simulink model "scara_stepper"  (R2026a)
settings: Solver=FixedStepDiscrete  StopTime=scara_ref.t(end)  FixedStep=scara_p.dt
InitFcn:
  | addpath(fileparts(fileparts(fileparts(get_param(bdroot,'FileName'))))); startup_scara(); if ~exist('scara_steps_signal','var') || ~exist('scara_ref','var') || ~isfield(scara_ref,'steps'), scara_setup('flower'); end
undefined symbols (not defined in the file): scara_p, scara_q0, scara_ref
libraries: simulink x14
settings Model: Creator=vutua  LastModifiedBy=vutua

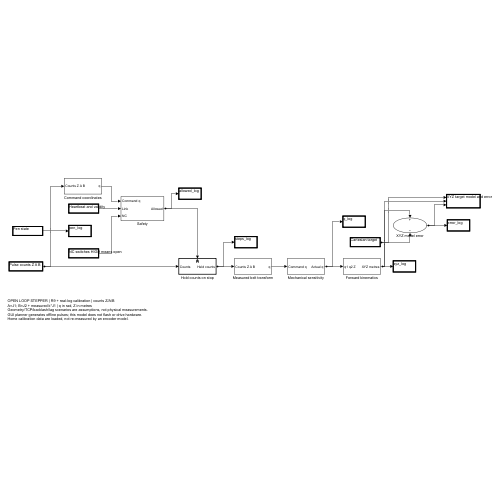
[thumbnail: Simulink's stored preview of the top-level diagram]
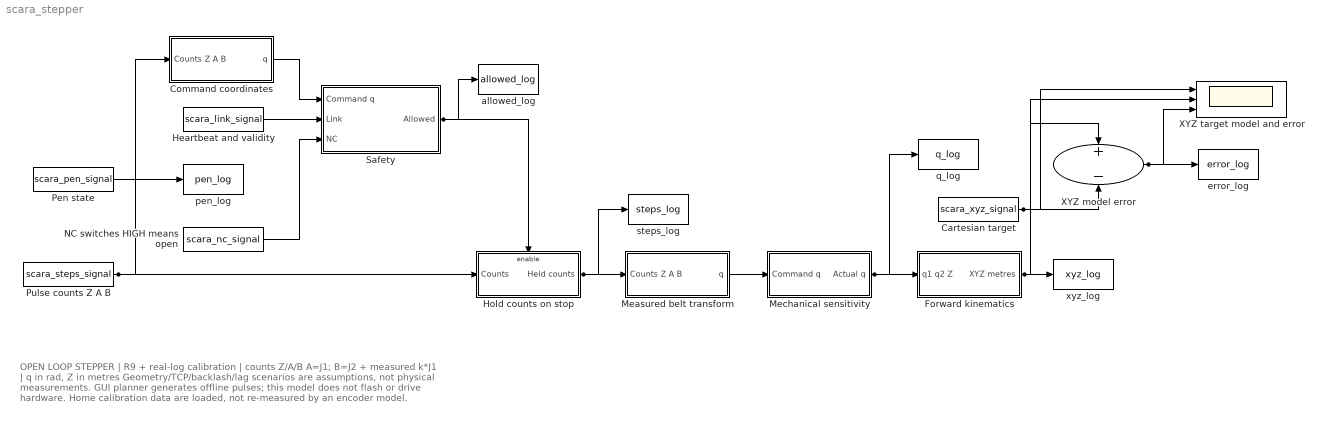
== system scara_stepper ==
  note: OPEN LOOP STEPPER | R9 + real-log calibration | counts Z/A/B
      | A=J1; B=J2 + measured k*J1 | q in rad, Z in metres
      | Geometry/TCP/backlash/lag scenarios are assumptions, not physical measurements.
      | GUI planner generates offline pulses; this model does not flash or drive hardware.
      | Home calibration data are loaded, not re-measured by an encoder model.
  Cartesian target : FromWorkspace  VariableName=scara_xyz_signal  SampleTime=scara_p.dt  Interpolate=off  OutputAfterFinalValue=Holding final value
  Command coordinates : Subsystem
  Forward kinematics : Subsystem
  Heartbeat and validity : FromWorkspace  VariableName=scara_link_signal  SampleTime=scara_p.dt  Interpolate=off  OutputAfterFinalValue=Holding final value
  Hold counts on stop : Subsystem
  Measured belt transform : Subsystem
  Mechanical sensitivity : Subsystem
  NC switches HIGH means open : FromWorkspace  VariableName=scara_nc_signal  SampleTime=scara_p.dt  Interpolate=off  OutputAfterFinalValue=Holding final value
  Pen state : FromWorkspace  VariableName=scara_pen_signal  SampleTime=scara_p.dt  Interpolate=off  OutputAfterFinalValue=Holding final value
  Pulse counts Z A B : FromWorkspace  VariableName=scara_steps_signal  SampleTime=scara_p.dt  Interpolate=off  OutputAfterFinalValue=Holding final value
  Safety : Subsystem
  XYZ model error : Sum  Inputs=+-
  XYZ target model and error : Scope  NumInputPorts=3
  allowed_log : ToWorkspace  VariableName=allowed_log  SampleTime=-1
  error_log : ToWorkspace  VariableName=error_log  SampleTime=-1
  pen_log : ToWorkspace  VariableName=pen_log  SampleTime=-1
  q_log : ToWorkspace  VariableName=q_log  SampleTime=-1
  steps_log : ToWorkspace  VariableName=steps_log  SampleTime=-1
  xyz_log : ToWorkspace  VariableName=xyz_log  SampleTime=-1
  wires:
  NC switches HIGH means open/1 -> Safety/3(NC)
  Command coordinates/1(q) -> Safety/1(Command q)
  Pulse counts Z A B/1 -> Hold counts on stop/1(Counts), Command coordinates/1(Counts Z A B)
  Pen state/1 -> pen_log/1
  Heartbeat and validity/1 -> Safety/2(Link)
  Hold counts on stop/1(Held counts) -> Measured belt transform/1(Counts Z A B), steps_log/1
  Safety/1(Allowed) -> allowed_log/1, Hold counts on stop/Enable
  Measured belt transform/1(q) -> Mechanical sensitivity/1(Command q)
  Forward kinematics/1(XYZ metres) -> XYZ model error/1, XYZ target model and error/2, xyz_log/1
  Mechanical sensitivity/1(Actual q) -> Forward kinematics/1(q1 q2 Z), q_log/1
  Cartesian target/1 -> XYZ model error/2, XYZ target model and error/1
  XYZ model error/1 -> error_log/1, XYZ target model and error/3

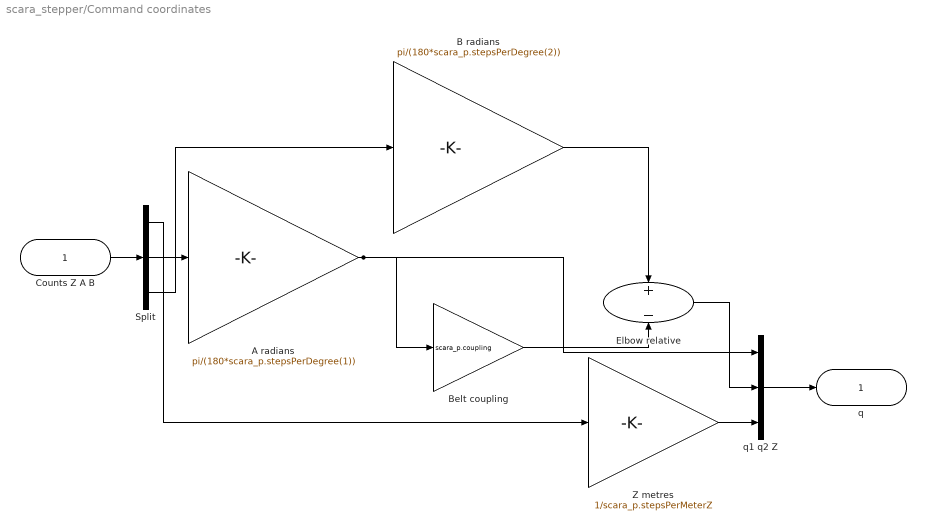
== system scara_stepper/Command coordinates ==
  Counts Z A B : Inport
  A radians : Gain  Gain=pi/(180*scara_p.stepsPerDegree(1))
  B radians : Gain  Gain=pi/(180*scara_p.stepsPerDegree(2))
  Belt coupling : Gain  Gain=scara_p.coupling
  Elbow relative : Sum  Inputs=+-
  Split : Demux  Outputs=3
  Z metres : Gain  Gain=1/scara_p.stepsPerMeterZ
  q1 q2 Z : Mux  Inputs=3
  q : Outport
  wires:
  Counts Z A B/1 -> Split/1
  B radians/1 -> Elbow relative/1
  Split/1 -> Z metres/1
  Split/2 -> A radians/1
  A radians/1 -> q1 q2 Z/1, Belt coupling/1
  Split/3 -> B radians/1
  Belt coupling/1 -> Elbow relative/2
  Elbow relative/1 -> q1 q2 Z/2
  Z metres/1 -> q1 q2 Z/3
  q1 q2 Z/1 -> q/1

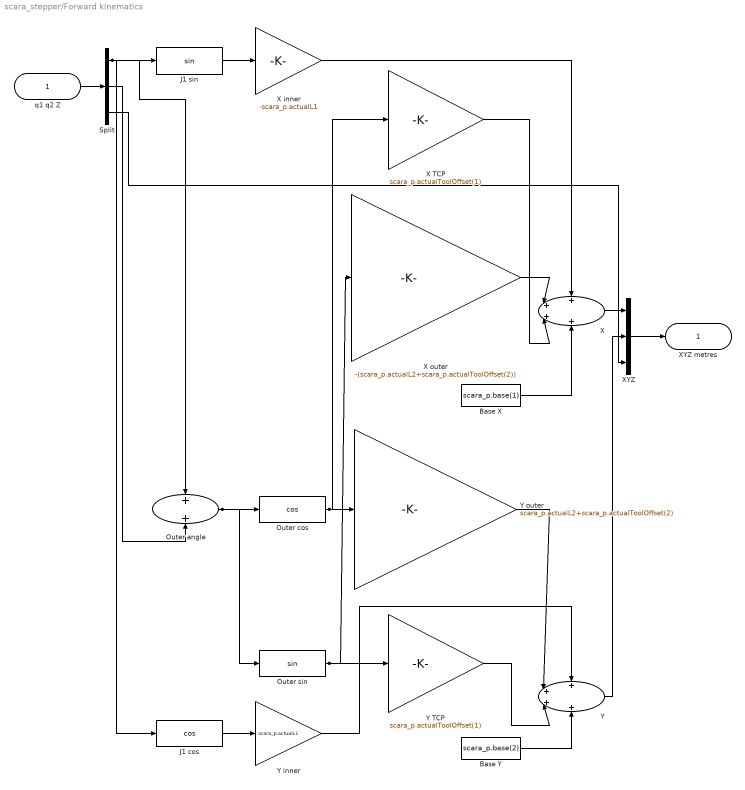
== system scara_stepper/Forward kinematics ==
  q1 q2 Z : Inport
  Base X : Constant  Value=scara_p.base(1)
  Base Y : Constant  Value=scara_p.base(2)
  J1 cos : Trigonometry  Operator=cos
  J1 sin : Trigonometry
  Outer angle : Sum
  Outer cos : Trigonometry  Operator=cos
  Outer sin : Trigonometry
  Split : Demux  Outputs=3
  X : Sum  Inputs=++++
  X TCP : Gain  Gain=scara_p.actualToolOffset(1)
  X inner : Gain  Gain=-scara_p.actualL1
  X outer : Gain  Gain=-(scara_p.actualL2+scara_p.actualToolOffset(2))
  XYZ : Mux  Inputs=3
  Y : Sum  Inputs=++++
  Y TCP : Gain  Gain=scara_p.actualToolOffset(1)
  Y inner : Gain  Gain=scara_p.actualL1
  Y outer : Gain  Gain=scara_p.actualL2+scara_p.actualToolOffset(2)
  XYZ metres : Outport
  wires:
  q1 q2 Z/1 -> Split/1
  X outer/1 -> X/2
  Split/1 -> Outer angle/1, J1 sin/1, J1 cos/1
  X inner/1 -> X/1
  J1 sin/1 -> X inner/1
  Split/2 -> Outer angle/2
  Split/3 -> XYZ/3
  Outer angle/1 -> Outer sin/1, Outer cos/1
  J1 cos/1 -> Y inner/1
  Outer cos/1 -> X TCP/1, Y outer/1
  Outer sin/1 -> X outer/1, Y TCP/1
  Y inner/1 -> Y/1
  X TCP/1 -> X/3
  Base X/1 -> X/4
  Y outer/1 -> Y/2
  Y TCP/1 -> Y/3
  XYZ/1 -> XYZ metres/1
  Base Y/1 -> Y/4
  X/1 -> XYZ/1
  Y/1 -> XYZ/2

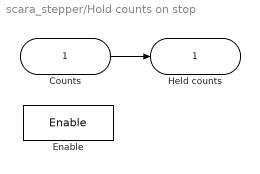
== system scara_stepper/Hold counts on stop ==
  Counts : Inport
  Enable : EnablePort
  Held counts : Outport  InitialOutput=scara_ref.steps(1,:)
  wires:
  Counts/1 -> Held counts/1

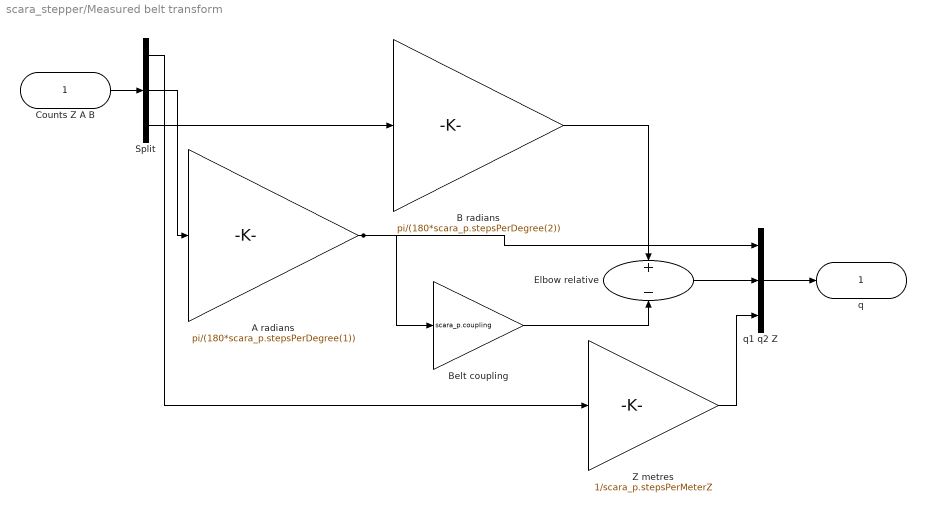
== system scara_stepper/Measured belt transform ==
  Counts Z A B : Inport
  A radians : Gain  Gain=pi/(180*scara_p.stepsPerDegree(1))
  B radians : Gain  Gain=pi/(180*scara_p.stepsPerDegree(2))
  Belt coupling : Gain  Gain=scara_p.coupling
  Elbow relative : Sum  Inputs=+-
  Split : Demux  Outputs=3
  Z metres : Gain  Gain=1/scara_p.stepsPerMeterZ
  q1 q2 Z : Mux  Inputs=3
  q : Outport
  wires:
  B radians/1 -> Elbow relative/1
  Counts Z A B/1 -> Split/1
  Belt coupling/1 -> Elbow relative/2
  Split/1 -> Z metres/1
  Split/2 -> A radians/1
  q1 q2 Z/1 -> q/1
  Elbow relative/1 -> q1 q2 Z/2
  A radians/1 -> Belt coupling/1, q1 q2 Z/1
  Split/3 -> B radians/1
  Z metres/1 -> q1 q2 Z/3

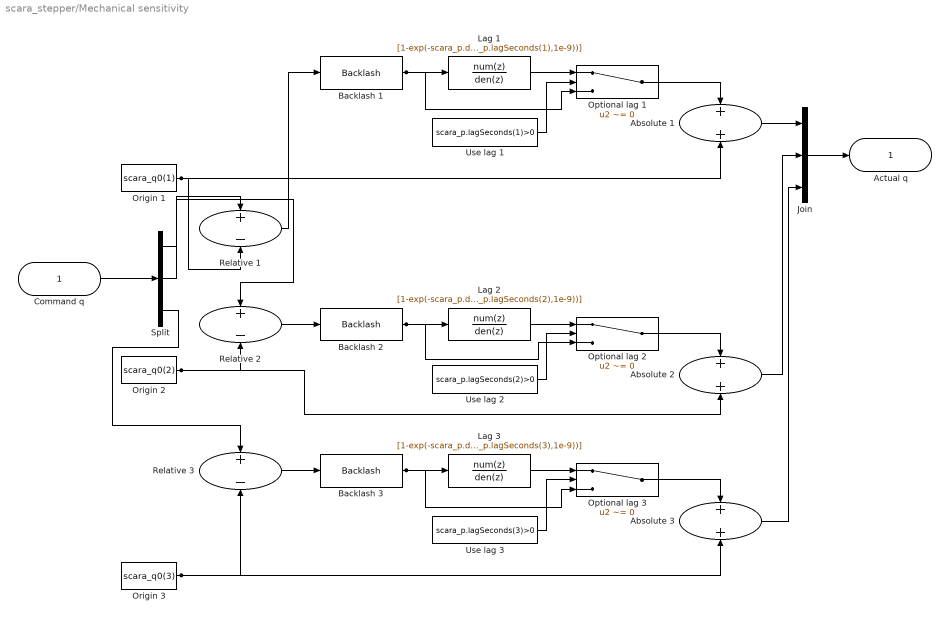
== system scara_stepper/Mechanical sensitivity ==
  Command q : Inport
  Absolute 1 : Sum
  Absolute 2 : Sum
  Absolute 3 : Sum
  Backlash 1 : Backlash  BacklashWidth=scara_p.backlash(1)  SampleTime=scara_p.dt
  Backlash 2 : Backlash  BacklashWidth=scara_p.backlash(2)  SampleTime=scara_p.dt
  Backlash 3 : Backlash  BacklashWidth=scara_p.backlash(3)  SampleTime=scara_p.dt
  Join : Mux  Inputs=3
  Lag 1 : DiscreteTransferFcn  Numerator=[1-exp(-scara_p.dt/max(scara_p.lagSeconds(1),1e-9)) 0]  Denominator=[1 -exp(-scara_p.dt/max(scara_p.lagSeconds(1),1e-9))]  SampleTime=scara_p.dt
  Lag 2 : DiscreteTransferFcn  Numerator=[1-exp(-scara_p.dt/max(scara_p.lagSeconds(2),1e-9)) 0]  Denominator=[1 -exp(-scara_p.dt/max(scara_p.lagSeconds(2),1e-9))]  SampleTime=scara_p.dt
  Lag 3 : DiscreteTransferFcn  Numerator=[1-exp(-scara_p.dt/max(scara_p.lagSeconds(3),1e-9)) 0]  Denominator=[1 -exp(-scara_p.dt/max(scara_p.lagSeconds(3),1e-9))]  SampleTime=scara_p.dt
  Optional lag 1 : Switch  Criteria=u2 ~= 0  SaturateOnIntegerOverflow=off  InputSameDT=off
  Optional lag 2 : Switch  Criteria=u2 ~= 0  SaturateOnIntegerOverflow=off  InputSameDT=off
  Optional lag 3 : Switch  Criteria=u2 ~= 0  SaturateOnIntegerOverflow=off  InputSameDT=off
  Origin 1 : Constant  Value=scara_q0(1)
  Origin 2 : Constant  Value=scara_q0(2)
  Origin 3 : Constant  Value=scara_q0(3)
  Relative 1 : Sum  Inputs=+-
  Relative 2 : Sum  Inputs=+-
  Relative 3 : Sum  Inputs=+-
  Split : Demux  Outputs=3
  Use lag 1 : Constant  Value=scara_p.lagSeconds(1)>0
  Use lag 2 : Constant  Value=scara_p.lagSeconds(2)>0
  Use lag 3 : Constant  Value=scara_p.lagSeconds(3)>0
  Actual q : Outport
  wires:
  Command q/1 -> Split/1
  Split/2 -> Relative 2/1
  Relative 1/1 -> Backlash 1/1
  Split/3 -> Relative 3/1
  Origin 2/1 -> Relative 2/2, Absolute 2/2
  Origin 1/1 -> Relative 1/2, Absolute 1/2
  Split/1 -> Relative 1/1
  Origin 3/1 -> Relative 3/2, Absolute 3/2
  Relative 2/1 -> Backlash 2/1
  Relative 3/1 -> Backlash 3/1
  Backlash 1/1 -> Optional lag 1/3, Lag 1/1
  Backlash 2/1 -> Optional lag 2/3, Lag 2/1
  Backlash 3/1 -> Optional lag 3/3, Lag 3/1
  Lag 1/1 -> Optional lag 1/1
  Use lag 1/1 -> Optional lag 1/2
  Lag 2/1 -> Optional lag 2/1
  Use lag 2/1 -> Optional lag 2/2
  Lag 3/1 -> Optional lag 3/1
  Use lag 3/1 -> Optional lag 3/2
  Optional lag 1/1 -> Absolute 1/1
  Absolute 2/1 -> Join/2
  Optional lag 2/1 -> Absolute 2/1
  Absolute 3/1 -> Join/3
  Optional lag 3/1 -> Absolute 3/1
  Absolute 1/1 -> Join/1
  Join/1 -> Actual q/1

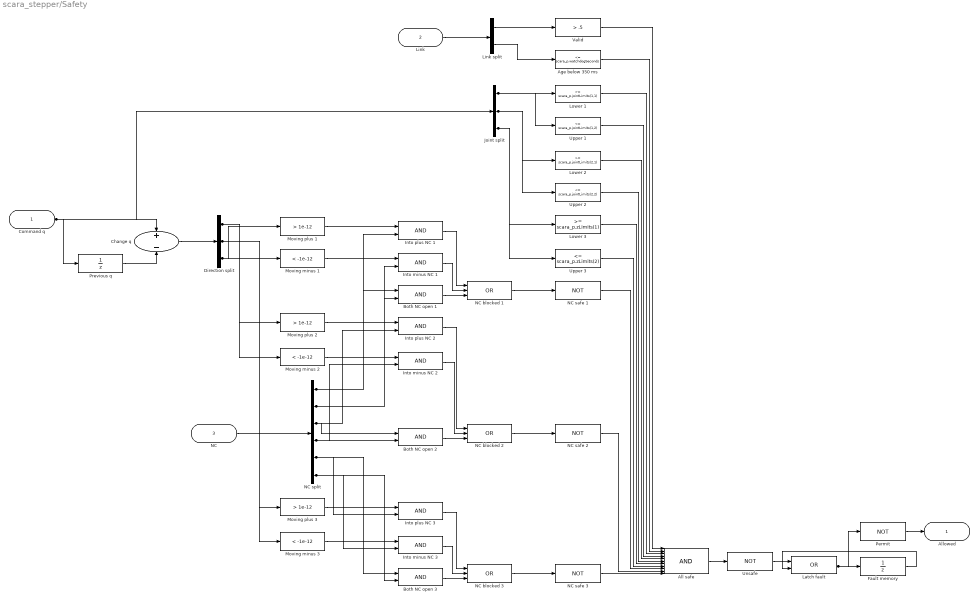
== system scara_stepper/Safety ==
  Command q : Inport
  Link : Inport  Port=2
  NC : Inport  Port=3
  Age below 350 ms : simulink/Logic and Bit Operations/Compare To Constant  relop=<=  const=scara_p.watchdogSeconds  OutDataTypeStr=boolean
  All safe : Logic  Inputs=11  AllPortsSameDT=off  OutDataTypeStr=boolean
  Both NC open 1 : Logic  AllPortsSameDT=off  OutDataTypeStr=boolean
  Both NC open 2 : Logic  AllPortsSameDT=off  OutDataTypeStr=boolean
  Both NC open 3 : Logic  AllPortsSameDT=off  OutDataTypeStr=boolean
  Change q : Sum  Inputs=+-
  Direction split : Demux  Outputs=3
  Fault memory : UnitDelay  SampleTime=scara_p.dt
  Into minus NC 1 : Logic  AllPortsSameDT=off  OutDataTypeStr=boolean
  Into minus NC 2 : Logic  AllPortsSameDT=off  OutDataTypeStr=boolean
  Into minus NC 3 : Logic  AllPortsSameDT=off  OutDataTypeStr=boolean
  Into plus NC 1 : Logic  AllPortsSameDT=off  OutDataTypeStr=boolean
  Into plus NC 2 : Logic  AllPortsSameDT=off  OutDataTypeStr=boolean
  Into plus NC 3 : Logic  AllPortsSameDT=off  OutDataTypeStr=boolean
  Joint split : Demux  Outputs=3
  Latch fault : Logic  Operator=OR  AllPortsSameDT=off  OutDataTypeStr=boolean
  Link split : Demux  Outputs=2
  Lower 1 : simulink/Logic and Bit Operations/Compare To Constant  relop=>=  const=scara_p.jointLimits(1,1)  OutDataTypeStr=boolean
  Lower 2 : simulink/Logic and Bit Operations/Compare To Constant  relop=>=  const=scara_p.jointLimits(2,1)  OutDataTypeStr=boolean
  Lower 3 : simulink/Logic and Bit Operations/Compare To Constant  relop=>=  const=scara_p.zLimits(1)  OutDataTypeStr=boolean
  Moving minus 1 : simulink/Logic and Bit Operations/Compare To Constant  relop=<  const=-1e-12  OutDataTypeStr=boolean
  Moving minus 2 : simulink/Logic and Bit Operations/Compare To Constant  relop=<  const=-1e-12  OutDataTypeStr=boolean
  Moving minus 3 : simulink/Logic and Bit Operations/Compare To Constant  relop=<  const=-1e-12  OutDataTypeStr=boolean
  Moving plus 1 : simulink/Logic and Bit Operations/Compare To Constant  relop=>  const=1e-12  OutDataTypeStr=boolean
  Moving plus 2 : simulink/Logic and Bit Operations/Compare To Constant  relop=>  const=1e-12  OutDataTypeStr=boolean
  Moving plus 3 : simulink/Logic and Bit Operations/Compare To Constant  relop=>  const=1e-12  OutDataTypeStr=boolean
  NC blocked 1 : Logic  Operator=OR  Inputs=3  AllPortsSameDT=off  OutDataTypeStr=boolean
  NC blocked 2 : Logic  Operator=OR  Inputs=3  AllPortsSameDT=off  OutDataTypeStr=boolean
  NC blocked 3 : Logic  Operator=OR  Inputs=3  AllPortsSameDT=off  OutDataTypeStr=boolean
  NC safe 1 : Logic  Operator=NOT  AllPortsSameDT=off  OutDataTypeStr=boolean
  NC safe 2 : Logic  Operator=NOT  AllPortsSameDT=off  OutDataTypeStr=boolean
  NC safe 3 : Logic  Operator=NOT  AllPortsSameDT=off  OutDataTypeStr=boolean
  NC split : Demux  Outputs=6
  Permit : Logic  Operator=NOT  AllPortsSameDT=off  OutDataTypeStr=boolean
  Previous q : UnitDelay  InitialCondition=scara_q0  SampleTime=scara_p.dt
  Unsafe : Logic  Operator=NOT  AllPortsSameDT=off  OutDataTypeStr=boolean
  Upper 1 : simulink/Logic and Bit Operations/Compare To Constant  relop=<=  const=scara_p.jointLimits(1,2)  OutDataTypeStr=boolean
  Upper 2 : simulink/Logic and Bit Operations/Compare To Constant  relop=<=  const=scara_p.jointLimits(2,2)  OutDataTypeStr=boolean
  Upper 3 : simulink/Logic and Bit Operations/Compare To Constant  relop=<=  const=scara_p.zLimits(2)  OutDataTypeStr=boolean
  Valid : simulink/Logic and Bit Operations/Compare To Constant  relop=>  const=.5  OutDataTypeStr=boolean
  Allowed : Outport
  wires:
  Command q/1 -> Joint split/1, Change q/1, Previous q/1
  Previous q/1 -> Change q/2
  Upper 2/1 -> All safe/6
  Moving plus 1/1 -> Into plus NC 1/1
  Joint split/2 -> Lower 2/1, Upper 2/1
  Direction split/2 -> Moving plus 3/1, Moving minus 3/1
  Lower 2/1 -> All safe/5
  Change q/1 -> Direction split/1
  Direction split/1 -> Moving plus 2/1, Moving minus 2/1
  NC split/5 -> Into plus NC 3/2, Both NC open 3/1
  NC/1 -> NC split/1
  Direction split/3 -> Moving plus 1/1, Moving minus 1/1
  Moving minus 1/1 -> Into minus NC 1/1
  Moving plus 2/1 -> Into plus NC 2/1
  Moving minus 2/1 -> Into minus NC 2/1
  NC split/1 -> Both NC open 1/1, Into plus NC 1/2
  NC split/2 -> Into minus NC 1/2, Both NC open 1/2
  NC split/3 -> Into plus NC 2/2, Both NC open 2/1
  NC split/4 -> Into minus NC 2/2, Both NC open 2/2
  Into plus NC 1/1 -> NC blocked 1/1
  NC split/6 -> Both NC open 3/2, Into minus NC 3/2
  Permit/1 -> Allowed/1
  Moving plus 3/1 -> Into plus NC 3/1
  Moving minus 3/1 -> Into minus NC 3/1
  Lower 3/1 -> All safe/7
  Link/1 -> Link split/1
  Into minus NC 1/1 -> NC blocked 1/2
  Into minus NC 2/1 -> NC blocked 2/2
  Both NC open 1/1 -> NC blocked 1/3
  Joint split/3 -> Lower 3/1, Upper 3/1
  Into minus NC 3/1 -> NC blocked 3/2
  Both NC open 2/1 -> NC blocked 2/3
  Into plus NC 2/1 -> NC blocked 2/1
  Upper 1/1 -> All safe/4
  Joint split/1 -> Lower 1/1, Upper 1/1
  Both NC open 3/1 -> NC blocked 3/3
  Into plus NC 3/1 -> NC blocked 3/1
  Latch fault/1 -> Fault memory/1, Permit/1
  Link split/1 -> Valid/1
  Link split/2 -> Age below 350 ms/1
  NC blocked 1/1 -> NC safe 1/1
  Age below 350 ms/1 -> All safe/2
  NC blocked 2/1 -> NC safe 2/1
  NC blocked 3/1 -> NC safe 3/1
  NC safe 2/1 -> All safe/10
  Valid/1 -> All safe/1
  Lower 1/1 -> All safe/3
  Upper 3/1 -> All safe/8
  NC safe 1/1 -> All safe/9
  NC safe 3/1 -> All safe/11
  All safe/1 -> Unsafe/1
  Unsafe/1 -> Latch fault/1
  Fault memory/1 -> Latch fault/2
